simulink model "fm_nfm"  (R2018a)
settings: Solver=ode45  StartTime=0.0  StopTime=0.5  RelTol=1e-3  EnableMultiTasking=on
PreLoadFcn:
  | %%%%%%%%%%%%%%%%%%%%%%%%%%%%%%%%%%%%%%%%%%%%%%%%%%%%%%%%%%%%%%%%%%%%%%%%%%%
  | % check to see if Simulink library folder is missing from the MATLAB path %
  | %%%%%%%%%%%%%%%%%%%%%%%%%%%%%%%%%%%%%%%%%%%%%%%%%%%%%%%%%%%%%%%%%%%%%%%%%%%
  | if isempty(strfind(path, 'rtlsdr_book_library'))
  | 
  |     % create error window
  |     fig_error = figure(...
  |         'Name', 'Error: RTL-SDR Book Library',...
  |         'Toolbar','none',...
  |         'MenuBar','none',...
  |         'NumberTitle','off',...
  |         'Resize','off',...
  |         'WindowStyle','modal');
  |     fig_error.Position(3) = 600;
  |     fig_error.Position(4) = 150;
  |     fig_axes = axes(...
  |         'Parent',fig_error,...
  |         'Position',[0,0,1,1],...
  |         'visible','off');
  |     % error message
  |     t_title = text(.05,.8,...
  |         'MISSING DIRECTORIES',...
  |         'FontSize',11.5);
  |     t_body = text(.075,.6,...
  |         [{'Simulink cannot find the  \it{<root>}\rm / \it{rtlsdr\_book\_library}\rm  folder in the \it{MATLAB Path}\rm.'},...
  |         {'Please set the MATLAB path following the instructions given in Exercise 2.4.'}],...
  |         'FontSize',10.5);
  |     % buttons
  |     btn_path = uicontrol(...
  |         'Parent',fig_error,...
  |         'String','Set Path Now',...
  |         'FontSize',10,...
  |         'Callback', 'pathtool; close(fig_error);',...
  |         'Position', [fig_error.Position(3)/2-210, 30, 200, 30]);
  |     btn_abort = uicontrol(...
  |         'Parent',fig_error,...
  |         'String','No thanks',...
  |         'FontSize',10,...
  |         'Callback', 'close(fig_error); abort=1;',...
  |         'Position', [fig_error.Position(3)/2+10, 30, 200, 30]);
  | 
  |     % pause to allow user to interact with error box
  |     uiwait(fig_error);
  | 
  |     % abort simulation
  |     try
  |         if abort==1
  |             set_param(gcs, 'SimulationCommand', 'stop');
  |         end
  |     end
  | 
  |     % if user has set path, allow diagram to be updated
  |     if ~exist('abort','var')
  |         % create error window
  |         fig_update = figure(...
  |             'Name', 'Update Diagram',...
  |             'Toolbar','none',...
  |             'MenuBar','none',...
  |             'NumberTitle','off',...
  |             'Resize','off');
  |         fig_update.Position(3) = 400;
  |         fig_update.Position(4) = 120;
  |         fig_axes = axes(...
  |             'Parent',fig_update,...
  |             'Position',[0,0,1,1],...
  |             'visible','off');
  |         % instruction message
  |         t_body = text(.075,.7,...
  |             'Once you have set the path, update the block diagram',...
  |             'FontSize',10.5);
  |         % button
  |         btn_update = uicontrol(...
  |             'Parent',fig_update,...
  |             'String','Update Block Diagram',...
  |             'FontSize',10,...
  |             'Callback', 'set_param(gcs,''SimulationCommand'',''update''); close(gcf)',...
  |             'Position', [fig_update.Position(3)/2-100, 30, 200, 30]);
  |     end
  | 
  |     % clear error components
  |     clear('fig_error','fig_update','fig_axes','t_title','t_body','btn_path','btn_abort','btn_update','abort');
  | 
  | end
  | %%%%%%%%%%%%%%%%%%%%%%%%%%%%%%%%%%%%%%%%%%%%%%%%%%%%%%%%%%%%%%%%%%%%%%%%%%%
PostLoadFcn:
  | fs  = 800e3;
  | 
  | singletone.Ai = 2;
  | singletone.fi = 2e3;
  | singletone.ph = 0;
  | 
  | bband1.Ai = 0.25;
  | bband1.fi = 1e3;
  | bband1.ph = pi/2;
  | 
  | bband2.Ai = 0.75;
  | bband2.fi = 2e3;
  | bband2.ph = 0;
  | 
  | bband3.Ai = 0.5;
  | bband3.fi = 3e3;
  | bband3.ph = pi/4;
  | 
  | bband4.Ai = 1.25;
  | bband4.fi = 4e3;
  | bband4.ph = pi/3;
  | 
  | carrier.Ac_single = 2;
  | carrier.Ac_sum  = 2;
  | carrier.fc = 50e3;
  | carrier.ph = 0;
  | 
  | Kvco_single =1e3;
  | Kvco_sum =1e3;
libraries: dspsrcs4 x2, commsynccomp2 x2
Description:
  | Software, Simulation Examples and Design Exercises Licence Agreement
  | 
  | This license agreement refers to the simulation examples, design exercises and files,
  | and associated software MATLAB and Simulink resources that accompany the book:
  | 
  |      Title: Software Defined Radio using MATLAB & Simulink and the RTL-SDR
  |      Published by Strathclyde Academic Media, 2015
  |      Authored by Robert W. Stewart, Kenneth W. Barlee, Dale S.W. Atkinson,
  |      and Louise H. Crockett
  | 
  | and made available as a download from, www.desktopSDR.com or variously acquired
  | by other means such as via USB storage, cloud storage, disk or any other electronic
  | or optical or magnetic storage mechanism. These files and associated software may
  | be used subject to the terms of agreement of the conditions below:
  | 
  |     Copyright © 2015 Robert W. Stewart, Kenneth W. Barlee, Dale S.W. Atkinson,
  |     and Louise H. Crockett
  |     All rights reserved.
  | 
  | Redistribution and use in source and binary forms, with or without modification, are
  | permitted provided that the following conditions are met:
  | 
  |    1.  Redistributions of source code must retain the above copyright notice, this list of
  |         conditions and the following disclaimer.
  | 
  |    2.  Redistributions in binary form must reproduce the above copyright notice, this
  |         list of conditions and the following disclaimer in the documentation and/or other
  |         materials provided with the distribution.
  | 
  |    3.  Neither the name of the copyright holder nor the names of its contributors may
  |         be used to endorse or promote products derived from this software without
  |         specific prior written permission.
  | 
  |    4.  In all cases, the software is, and all modifications and derivatives of the
  |         software shall be, licensed to you solely for use in conjunction with The
  |         MathWorks, Inc. products and service offerings.
  | 
  | THIS SOFTWARE IS PROVIDED BY THE COPYRIGHT HOLDERS AND CONTRIBUTORS
  | "AS IS" AND ANY EXPRESS OR IMPLIED WARRANTIES, INCLUDING, BUT NOT LIMITED
  | TO, THE IMPLIED WARRANTIES OF MERCHANTABILITY AND FITNESS FOR A
  | PARTICULAR PURPOSE ARE DISCLAIMED. IN NO EVENT SHALL THE COPYRIGHT
  | HOLDER OR CONTRIBUTORS BE LIABLE FOR ANY DIRECT, INDIRECT, INCIDENTAL,
  | SPECIAL, EXEMPLARY, OR CONSEQUENTIAL DAMAGES (INCLUDING, BUT NOT
  | LIMITED TO, PROCUREMENT OF SUBSTITUTE GOODS OR SERVICES; LOSS OF USE,
  | DATA, OR PROFITS; OR BUSINESS INTERRUPTION) HOWEVER CAUSED AND ON ANY
  | THEORY OF LIABILITY, WHETHER IN CONTRACT, STRICT LIABILITY, OR TORT
  | (INCLUDING NEGLIGENCE OR OTHERWISE) ARISING IN ANY WAY OUT OF THE USE
  | OF THIS SOFTWARE, EVEN IF ADVISED OF THE POSSIBILITY OF SUCH DAMAGE.
  | 
  | 
  | Audio Tracks used in Simulations Examples and Design Exercises
  | 
  | The music and vocal files used within the Examples files and software within the book
  | were variously written, arranged, performed, recorded and produced by Garrey Rice,
  | Adam Struth, Jamie Struth, Iain Thistlethwaite and also Marshall Craigmyle who
  | collectively, and individually where appropriate, assert and retain all of their copyright,
  | performance and artistic rights. Permission to use and reproduce this music is
  | granted for all purposes associated with MATLAB and Simulink software and the
  | simulation examples and design exercises files that accompany this book. Requests to
  | use the music for any other purpose should be directed to: info@desktopSDR.com.
  | For information on music track names, full credits, and links to the musicians please
  | refer to www.desktopSDR.com/more/audio.
settings Model: ModifiedByFormat=desktopSDR Team  Creator=desktopSDR Team  LastModifiedBy=desktopSDR Team
settings DataIOCC: SaveFormat=Array  SaveOutput=off  SignalLogging=off  SaveTime=off
settings OptimizationCC: LifeSpan=inf
settings DebuggingCC: SolverPrmCheckMsg=warning  SFUnexpectedBacktrackingDiag=warning  SFNoUnconditionalDefaultTransitionDiag=warning  SFExecutionAtInitializationDiag=none
settings HardwareCC: ProdBitPerPointer=32  ProdBitPerSizeT=32  ProdBitPerPtrDiffT=32  ProdLargestAtomicFloat=None  ProdIntDivRoundTo=Undefined  ProdEndianess=Unspecified  ProdWordSize=32  ProdHWDeviceType=32-bit Generic
settings ModelReferenceCC: PropagateSignalLabelsOutOfModel=off
settings CodeAppCC: StateflowObjectComments=on
settings GRTTargetCC: TargetLangStandard=C89/C90 (ANSI)  GeneratePreprocessorConditionals=Disable all
settings ConfigComp: CovMetricSettings=dw  CovHtmlReporting=on  CovSaveCumulativeToWorkspaceVar=on  CovSaveSingleToWorkspaceVar=on  CovExternalEMLEnable=off  CovSFcnEnable=off

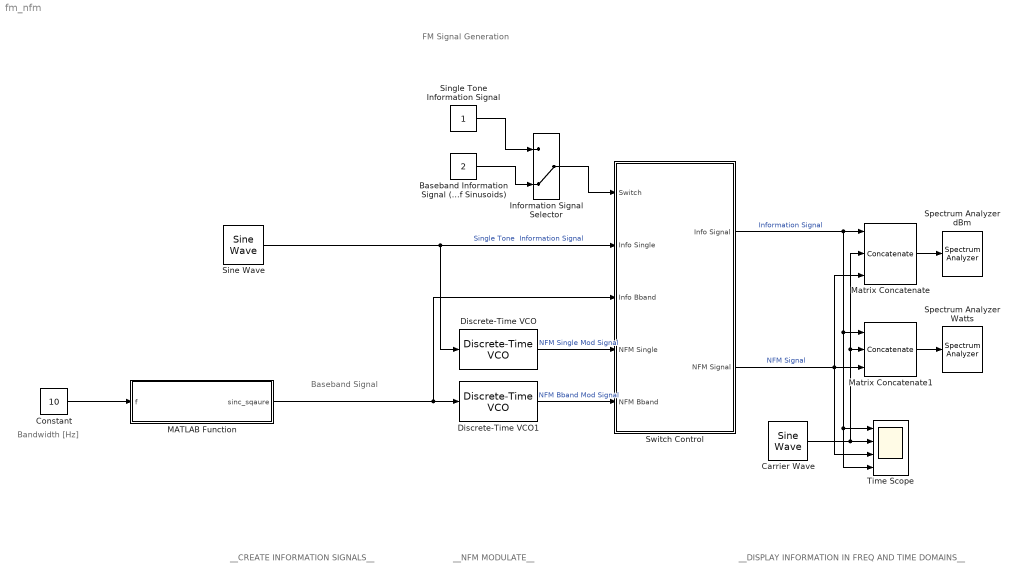
== system fm_nfm ==
  note: Baseband Signal
  note: Bandwidth [Hz]
  note: FM Signal Generation
  note: __CREATE INFORMATION SIGNALS__
  note: __NFM MODULATE__
  note: __DISPLAY INFORMATION IN FREQ AND TIME DOMAINS__
  Baseband Information Signal (Sum of Sinusoids) : Constant  Value=2
  Carrier Wave : dspsrcs4/Sine Wave  Amplitude=carrier.Ac_single  Frequency=carrier.fc  Phase=carrier.ph  SampleMode=Discrete  OutComplex=Real  CompMethod=Trigonometric fcn  TableSize=Speed  SampleTime=1/fs  SamplesPerFrame=1  ResetState=Restart at time zero  OutputFrames=on  dataType=double  wordLen=16  udDataType=sfix(16)  fracBitsMode=Best precision  numFracBits=15  OutDataTypeStr=double  LastOutDataTypeStr=double
  Constant : Constant  Value=10
  Discrete-Time VCO : commsynccomp2/Discrete-Time VCO  Ac=carrier.Ac_single  Fc=carrier.fc  Kc=Kvco_single  Ph=carrier.ph  ts=1/fs
      settings: SourceProductName=Communications System Toolbox  SourceProductBaseCode=CM
  Discrete-Time VCO1 : commsynccomp2/Discrete-Time VCO  Ac=carrier.Ac_sum  Fc=carrier.fc  Kc=Kvco_sum  Ph=carrier.ph  ts=1/fs
      settings: SourceProductName=Communications System Toolbox  SourceProductBaseCode=CM
  Information Signal Selector : ManualSwitch  CurrentSetting=0
  MATLAB Function : MATLAB Function  TreatAsAtomicUnit=on
  Matrix Concatenate : Concatenate  NumInputs=3  Mode=Multidimensional array  ConcatenateDimension=2
  Matrix Concatenate1 : Concatenate  NumInputs=3  Mode=Multidimensional array  ConcatenateDimension=2
  Sine Wave : dspsrcs4/Sine Wave  Amplitude=singletone.Ai  Frequency=singletone.fi  Phase=singletone.ph  SampleMode=Discrete  OutComplex=Real  CompMethod=Trigonometric fcn  TableSize=Speed  SampleTime=1/fs  SamplesPerFrame=1  ResetState=Restart at time zero  OutputFrames=on  dataType=double  wordLen=16  udDataType=sfix(16)  fracBitsMode=Best precision  numFracBits=15  OutDataTypeStr=double  LastOutDataTypeStr=double
  Single Tone Information Signal : Constant
  Spectrum Analyzer Watts : SpectrumAnalyzer
  Spectrum Analyzer dBm : SpectrumAnalyzer
  Switch Control : Subsystem
  Time Scope : Scope  NumInputPorts=4
  wires:
  Sine Wave/1 -> Discrete-Time VCO/1, Switch Control/2(Info Single)  "Single Tone  Information Signal"
  MATLAB Function/1(sinc_sqaure) -> Switch Control/3(Info Bband), Discrete-Time VCO1/1
  Switch Control/1(Info Signal) -> Matrix Concatenate/1, Time Scope/4, Time Scope/1, Matrix Concatenate1/1  "Information Signal"
  Carrier Wave/1 -> Matrix Concatenate/2, Matrix Concatenate1/2, Time Scope/2
  Switch Control/2(NFM Signal) -> Matrix Concatenate1/3, Matrix Concatenate/3, Time Scope/3  "NFM Signal"
  Matrix Concatenate1/1 -> Spectrum Analyzer Watts/1
  Information Signal Selector/1 -> Switch Control/1(Switch)
  Single Tone Information Signal/1 -> Information Signal Selector/1
  Baseband Information Signal (Sum of Sinusoids)/1 -> Information Signal Selector/2
  Discrete-Time VCO/1 -> Switch Control/4(NFM Single)  "NFM Single Mod Signal"
  Discrete-Time VCO1/1 -> Switch Control/5(NFM Bband)  "NFM Bband Mod Signal"
  Matrix Concatenate/1 -> Spectrum Analyzer dBm/1
  Constant/1 -> MATLAB Function/1(f)

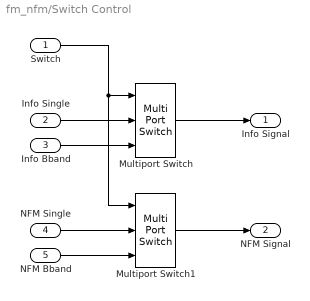
== system fm_nfm/Switch Control ==
  Switch : Inport
  Info Single : Inport  Port=2
  Info Bband : Inport  Port=3
  NFM Single : Inport  Port=4
  NFM Bband : Inport  Port=5
  Multiport Switch : MultiPortSwitch  Inputs=2
  Multiport Switch1 : MultiPortSwitch  Inputs=2
  Info Signal : Outport
  NFM Signal : Outport  Port=2
  wires:
  Multiport Switch1/1 -> NFM Signal/1
  Switch/1 -> Multiport Switch1/1, Multiport Switch/1
  Info Single/1 -> Multiport Switch/2
  Multiport Switch/1 -> Info Signal/1
  Info Bband/1 -> Multiport Switch/3
  NFM Single/1 -> Multiport Switch1/2
  NFM Bband/1 -> Multiport Switch1/3

== matlab function fm_nfm/MATLAB Function ==
  data: f input; sinc_sqaure output
function sinc_sqaure = fcn(f)


fs = 800e3; Ts = 1/fs ;

start_time = 0 ; end_time = 1 ; % in s;

t_sampled = start_time:Ts:end_time - Ts;

% f: bandwidth in Hz 

sinc_sqaure = f*((sinc(f*t_sampled)).^2);


end
